simulink model "ros2_autosar_bridge"  (R2022b)
settings: Solver=VariableStepAuto  StartTime=0.0  StopTime=10.0  RelTol=1e-3
libraries: ros2lib x9
settings Model: Creator=Mohamed Mehdi Hamdi  LastModifiedBy=Mohamed Mehdi Hamdi

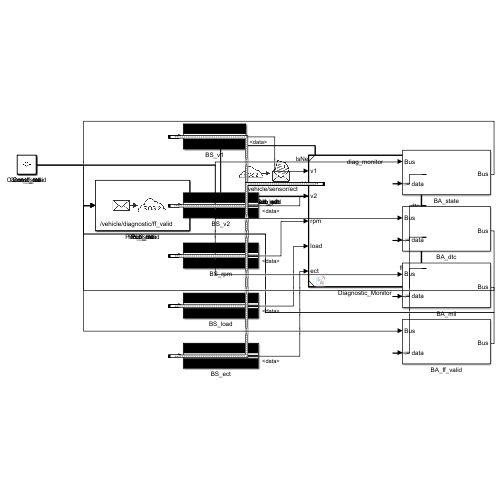
[thumbnail: Simulink's stored preview of the top-level diagram]
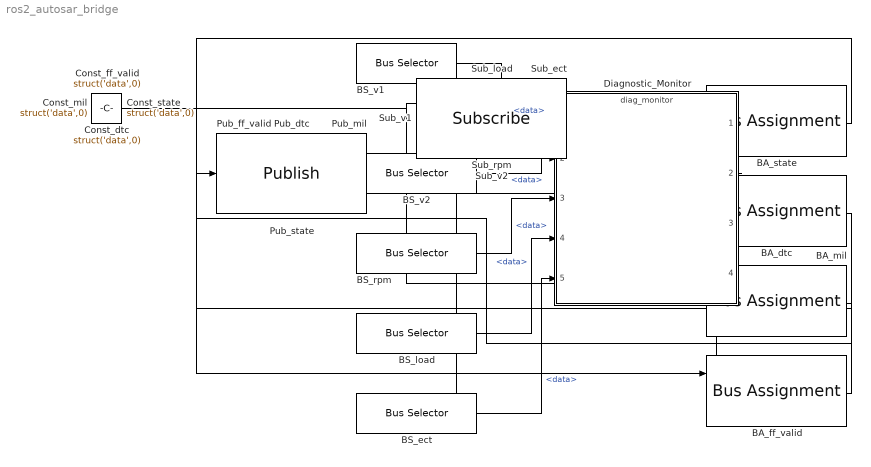
== system ros2_autosar_bridge ==
  BA_dtc : BusAssignment  AssignedSignals=data
  BA_ff_valid : BusAssignment  AssignedSignals=data
  BA_mil : BusAssignment  AssignedSignals=data
  BA_state : BusAssignment  AssignedSignals=data
  BS_ect : BusSelector  OutputSignals=data
  BS_load : BusSelector  OutputSignals=data
  BS_rpm : BusSelector  OutputSignals=data
  BS_v1 : BusSelector  OutputSignals=data
  BS_v2 : BusSelector  OutputSignals=data
  Const_dtc : Constant  Value=struct('data',0)  OutDataTypeStr=Bus: SL_Bus_std_msgs_UInt8
  Const_ff_valid : Constant  Value=struct('data',0)  OutDataTypeStr=Bus: SL_Bus_std_msgs_Bool
  Const_mil : Constant  Value=struct('data',0)  OutDataTypeStr=Bus: SL_Bus_std_msgs_Bool
  Const_state : Constant  Value=struct('data',0)  OutDataTypeStr=Bus: SL_Bus_std_msgs_UInt8
  Diagnostic_Monitor : ModelReference  ModelNameDialog=diag_monitor  SimulationMode=Normal  ModelReferenceVersion=1.1
  Pub_dtc : ros2lib/Publish  topicSource=Specify your own  topic=/vehicle/diagnostic/dtc  messageType=std_msgs/UInt8  QOSHistory=Keep last  QOSDepth=1  QOSReliability=Reliable  QOSDurability=Volatile
      settings: LibrarySourceBlock=roslib/ROS 2/Publish
  Pub_ff_valid : ros2lib/Publish  topicSource=Specify your own  topic=/vehicle/diagnostic/ff_valid  messageType=std_msgs/Bool  QOSHistory=Keep last  QOSDepth=1  QOSReliability=Reliable  QOSDurability=Volatile
      settings: LibrarySourceBlock=roslib/ROS 2/Publish
  Pub_mil : ros2lib/Publish  topicSource=Specify your own  topic=/vehicle/diagnostic/mil  messageType=std_msgs/Bool  QOSHistory=Keep last  QOSDepth=1  QOSReliability=Reliable  QOSDurability=Volatile
      settings: LibrarySourceBlock=roslib/ROS 2/Publish
  Pub_state : ros2lib/Publish  topicSource=Specify your own  topic=/vehicle/diagnostic/state  messageType=std_msgs/UInt8  QOSHistory=Keep last  QOSDepth=1  QOSReliability=Reliable  QOSDurability=Volatile
      settings: LibrarySourceBlock=roslib/ROS 2/Publish
  Sub_ect : ros2lib/Subscribe  topicSource=Specify your own  topic=/vehicle/sensor/ect  messageType=std_msgs/Float64  sampleTime=-1  QOSHistory=Keep last  QOSDepth=1  QOSReliability=Reliable  QOSDurability=Volatile
      settings: LibrarySourceBlock=roslib/ROS 2/Subscribe
  Sub_load : ros2lib/Subscribe  topicSource=Specify your own  topic=/vehicle/sensor/load  messageType=std_msgs/Float64  sampleTime=-1  QOSHistory=Keep last  QOSDepth=1  QOSReliability=Reliable  QOSDurability=Volatile
      settings: LibrarySourceBlock=roslib/ROS 2/Subscribe
  Sub_rpm : ros2lib/Subscribe  topicSource=Specify your own  topic=/vehicle/sensor/rpm  messageType=std_msgs/Float64  sampleTime=-1  QOSHistory=Keep last  QOSDepth=1  QOSReliability=Reliable  QOSDurability=Volatile
      settings: LibrarySourceBlock=roslib/ROS 2/Subscribe
  Sub_v1 : ros2lib/Subscribe  topicSource=Specify your own  topic=/vehicle/sensor/v1  messageType=std_msgs/Float64  sampleTime=-1  QOSHistory=Keep last  QOSDepth=1  QOSReliability=Reliable  QOSDurability=Volatile
      settings: LibrarySourceBlock=roslib/ROS 2/Subscribe
  Sub_v2 : ros2lib/Subscribe  topicSource=Specify your own  topic=/vehicle/sensor/v2  messageType=std_msgs/Float64  sampleTime=-1  QOSHistory=Keep last  QOSDepth=1  QOSReliability=Reliable  QOSDurability=Volatile
      settings: LibrarySourceBlock=roslib/ROS 2/Subscribe
  wires:
  Sub_v1/2 -> BS_v1/1
  BS_v1/1 -> Diagnostic_Monitor/1  "<data>"
  Sub_v2/2 -> BS_v2/1
  BS_v2/1 -> Diagnostic_Monitor/2  "<data>"
  Sub_rpm/2 -> BS_rpm/1
  BS_rpm/1 -> Diagnostic_Monitor/3  "<data>"
  Sub_load/2 -> BS_load/1
  BS_load/1 -> Diagnostic_Monitor/4  "<data>"
  Sub_ect/2 -> BS_ect/1
  BS_ect/1 -> Diagnostic_Monitor/5  "<data>"
  Const_state/1 -> BA_state/1
  Diagnostic_Monitor/1 -> BA_state/2
  BA_state/1 -> Pub_state/1
  Const_dtc/1 -> BA_dtc/1
  Diagnostic_Monitor/2 -> BA_dtc/2
  BA_dtc/1 -> Pub_dtc/1
  Const_mil/1 -> BA_mil/1
  Diagnostic_Monitor/3 -> BA_mil/2
  BA_mil/1 -> Pub_mil/1
  Const_ff_valid/1 -> BA_ff_valid/1
  Diagnostic_Monitor/4 -> BA_ff_valid/2
  BA_ff_valid/1 -> Pub_ff_valid/1
